simulink model "inverter_s2_kal"  (R2023b)
settings: Solver=ode15s  StartTime=0.0  StopTime=0.1  MaxStep=sim_max_step  RelTol=sim_rel_tol  AbsTol=sim_abs_tol  EnableMultiTasking=on
PreLoadFcn:
  | d08_pre_dir = fileparts(which('inverter_s2_kal')); if isempty(d08_pre_dir), d08_pre_dir = pwd; end; run(fullfile(d08_pre_dir, 'inverter_common_parameters.m')); clear d08_pre_dir
InitFcn:
  | run(fullfile(fileparts(get_param(bdroot,'FileName')),'inverter_common_parameters.m'));
  | kal_dosya = fullfile(fileparts(get_param(bdroot,'FileName')), [bdroot '_kalibrasyon.m']); if isfile(kal_dosya), run(kal_dosya); end; clear kal_dosya
values from neighbouring files (symbols this model uses):
  EMC_k = EMC_M/EMC_Lw    (= 0.995)    [inverter_common_parameters.m]
  EMC_Rcore = 1e5    (= 100000)    [inverter_common_parameters.m]
  EMC_Rw = 5e-3    (= 0.005)    [inverter_common_parameters.m]
  f_grid = 50    [inverter_common_parameters.m]
  K11 = 0.7865    [inverter_common_parameters.m]    (also in inverter_s1_kal_kalibrasyon.m = 0.7865023595)
  K12 = 0.79400    (= 0.794)    [inverter_common_parameters.m]    (also in inverter_s2_kal_kalibrasyon.m = 0.7679568)
  L1_core_Rp = 600    [inverter_common_parameters.m]
  measurement_gain = 20    [inverter_common_parameters.m]
  phase_deg1 = -0.44    [inverter_common_parameters.m]    (also in inverter_s1_kal_kalibrasyon.m = -0.36607)
  phase_deg2 = 0    [inverter_common_parameters.m]    (also in inverter_s2_kal_kalibrasyon.m = 0.1121)
  pwm_ref_amp = 1    [inverter_common_parameters.m]
  pwm_ref_Ts = 1e-6    (= 1e-06)    [inverter_common_parameters.m]
  R_bleed_1 = 220e3    (= 220000)    [inverter_common_parameters.m]
  R_bleed_2 = 220e3    (= 220000)    [inverter_common_parameters.m]
  Rdc = 1e-3    (= 0.001)    [inverter_common_parameters.m]
libraries: ee_lib x64, fl_lib x54, nesl_utility x30, spsOnDelayLib x12, spsMeanLib x10, spsPWMGeneratorDCDCLib x6, spsTHDLib x4, eePowerMeasurement x2, spsPowerLib x2, spsRMSLib x2, spspowerguiLib x1
(part 3 of 3)

== system inverter_s2_kal/AC Current Sensor1 ==
  Current Sensor : fl_lib/Electrical/Electrical Sensors/Current Sensor
  PS-Simulink Converter : nesl_utility/PS-Simulink Converter  PhysicalDomain=network_engine_domain  SubClassName=ps_output  LeftPortType=input  RightPortType=output  PseudoPeriodic=off  Frequencies=[]  VectorFormat=1-D array  Unit=1  AffineConversion=off
  + : PMIOPort  Side=Right
  - : PMIOPort  Port=2  Side=Right
  tag scope: i_ac1=global
  wires:
  PS-Simulink Converter/1 -> [i_ac1]
  connections:
  Current Sensor/RConn1 -- PS-Simulink Converter/LConn1
  +/RConn1 -- Current Sensor/LConn1
  Current Sensor/RConn2 -- -/RConn1

== system inverter_s2_kal/AC Current Sensor2 ==
  Current Sensor : fl_lib/Electrical/Electrical Sensors/Current Sensor
  PS-Simulink Converter : nesl_utility/PS-Simulink Converter  PhysicalDomain=network_engine_domain  SubClassName=ps_output  LeftPortType=input  RightPortType=output  PseudoPeriodic=off  Frequencies=[]  VectorFormat=1-D array  Unit=1  AffineConversion=off
  + : PMIOPort  Side=Right
  - : PMIOPort  Port=2  Side=Right
  tag scope: i_ac2=global
  wires:
  PS-Simulink Converter/1 -> [i_ac2]
  connections:
  Current Sensor/RConn1 -- PS-Simulink Converter/LConn1
  +/RConn1 -- Current Sensor/LConn1
  Current Sensor/RConn2 -- -/RConn1

== system inverter_s2_kal/AC Voltage Sensor1 ==
  PS-Simulink Converter : nesl_utility/PS-Simulink Converter  PhysicalDomain=network_engine_domain  SubClassName=ps_output  LeftPortType=input  RightPortType=output  PseudoPeriodic=off  Frequencies=[]  VectorFormat=1-D array  Unit=1  AffineConversion=off
  Voltage Sensor : fl_lib/Electrical/Electrical Sensors/Voltage Sensor
  - : PMIOPort  Side=Left
  + : PMIOPort  Port=2  Side=Right
  tag scope: v_ac1=global
  wires:
  PS-Simulink Converter/1 -> [v_ac1]
  connections:
  Voltage Sensor/RConn2 -- -/RConn1
  Voltage Sensor/RConn1 -- PS-Simulink Converter/LConn1
  Voltage Sensor/LConn1 -- +/RConn1

== system inverter_s2_kal/AC Voltage Sensor2 ==
  PS-Simulink Converter : nesl_utility/PS-Simulink Converter  PhysicalDomain=network_engine_domain  SubClassName=ps_output  LeftPortType=input  RightPortType=output  PseudoPeriodic=off  Frequencies=[]  VectorFormat=1-D array  Unit=1  AffineConversion=off
  Voltage Sensor : fl_lib/Electrical/Electrical Sensors/Voltage Sensor
  - : PMIOPort  Side=Left
  + : PMIOPort  Port=2  Side=Right
  tag scope: v_inv1=global
  wires:
  PS-Simulink Converter/1 -> [v_inv1]
  connections:
  Voltage Sensor/LConn1 -- +/RConn1
  Voltage Sensor/RConn1 -- PS-Simulink Converter/LConn1
  Voltage Sensor/RConn2 -- -/RConn1

== system inverter_s2_kal/AC Voltage Sensor3 ==
  PS-Simulink Converter : nesl_utility/PS-Simulink Converter  PhysicalDomain=network_engine_domain  SubClassName=ps_output  LeftPortType=input  RightPortType=output  PseudoPeriodic=off  Frequencies=[]  VectorFormat=1-D array  Unit=1  AffineConversion=off
  Voltage Sensor : fl_lib/Electrical/Electrical Sensors/Voltage Sensor
  - : PMIOPort  Side=Left
  + : PMIOPort  Port=2  Side=Right
  tag scope: v_ac2=global
  wires:
  PS-Simulink Converter/1 -> [v_ac2]
  connections:
  Voltage Sensor/RConn2 -- -/RConn1
  Voltage Sensor/RConn1 -- PS-Simulink Converter/LConn1
  Voltage Sensor/LConn1 -- +/RConn1

== system inverter_s2_kal/AC Voltage Sensor4 ==
  PS-Simulink Converter : nesl_utility/PS-Simulink Converter  PhysicalDomain=network_engine_domain  SubClassName=ps_output  LeftPortType=input  RightPortType=output  PseudoPeriodic=off  Frequencies=[]  VectorFormat=1-D array  Unit=1  AffineConversion=off
  Voltage Sensor : fl_lib/Electrical/Electrical Sensors/Voltage Sensor
  - : PMIOPort  Side=Left
  + : PMIOPort  Port=2  Side=Right
  tag scope: v_inv2=global
  wires:
  PS-Simulink Converter/1 -> [v_inv2]
  connections:
  Voltage Sensor/LConn1 -- +/RConn1
  Voltage Sensor/RConn1 -- PS-Simulink Converter/LConn1
  Voltage Sensor/RConn2 -- -/RConn1

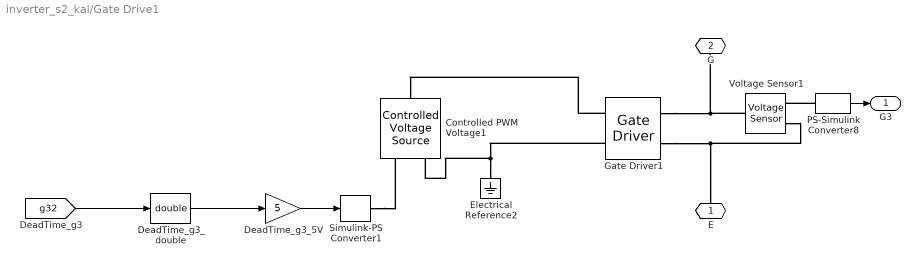
== system inverter_s2_kal/Gate Drive1 ==
  Controlled PWM Voltage1 : fl_lib/Electrical/Electrical Sources/Controlled Voltage Source
  DeadTime_g3_5V : Gain  Gain=5  OutDataTypeStr=double
  DeadTime_g3_double : DataTypeConversion  OutDataTypeStr=double  SaturateOnIntegerOverflow=off  RndMeth=Floor
  Electrical Reference2 : fl_lib/Electrical/Electrical Elements/Electrical Reference
  Gate Driver1 : ee_lib/Semiconductors & Converters/Gate Driver  port_option=ee.enum.controlport.elec  uHigh=4 V  uLow=3 V  uHighValue=gate_logic_high  uLowValue=gate_logic_low  vHigh=Vgate_on V  vLow=Vgate_off V  tHigh=gate_driver_ton s  tLow=gate_driver_toff s  parameterization=1  rHigh=RG_total Ohm  rLow=RG_total Ohm  tRise=gate_driver_rise s  tFall=gate_driver_fall s  cLoad=gate_driver_cload F  enable_faults=0  t_fault=1 s  fault_type=1  ZonTime_specify=off  ZonTime_priority=None  ZonTime=0 s  ZoffTime_specify=off  ZoffTime_priority=None  ZoffTime=0 s
  PS-Simulink Converter8 : nesl_utility/PS-Simulink Converter  PhysicalDomain=network_engine_domain  SubClassName=ps_output  LeftPortType=input  RightPortType=output  PseudoPeriodic=off  Frequencies=[]  VectorFormat=1-D array  Unit=1  AffineConversion=off
  Simulink-PS Converter1 : nesl_utility/Simulink-PS Converter  PhysicalDomain=network_engine_domain  SubClassName=ps_input  LeftPortType=input  RightPortType=output  PseudoPeriodic=off  Frequencies=[]  NoiseDistribution=none  NoiseParameters=[]  Unit=V  AffineConversion=off  FilteringAndDerivatives=filter  SimscapeFilterOrder=1  InputFilterTimeConstant=1e-7  UdotUserProvided=1
  Voltage Sensor1 : fl_lib/Electrical/Electrical Sensors/Voltage Sensor
  E : PMIOPort  Side=Right
  G : PMIOPort  Port=2  Side=Right
  G3 : Outport  VectorParamsAs1DForOutWhenUnconnected=off
  wires:
  PS-Simulink Converter8/1 -> G3/1
  [g32] -> DeadTime_g3_double/1
  DeadTime_g3_double/1 -> DeadTime_g3_5V/1
  DeadTime_g3_5V/1 -> Simulink-PS Converter1/1
  connections:
  Gate Driver1/RConn2 -- Voltage Sensor1/RConn2 -- E/RConn1
  Gate Driver1/RConn1 -- Voltage Sensor1/LConn1 -- G/RConn1
  PS-Simulink Converter8/LConn1 -- Voltage Sensor1/RConn1
  Gate Driver1/LConn2 -- Electrical Reference2/LConn1 -- Controlled PWM Voltage1/RConn2
  Simulink-PS Converter1/RConn1 -- Controlled PWM Voltage1/RConn1
  Gate Driver1/LConn1 -- Controlled PWM Voltage1/LConn1

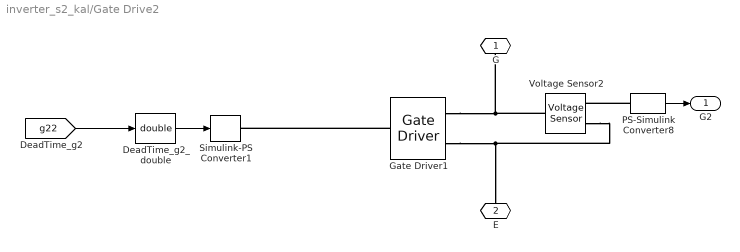
== system inverter_s2_kal/Gate Drive2 ==
  DeadTime_g2_double : DataTypeConversion  OutDataTypeStr=double  SaturateOnIntegerOverflow=off  RndMeth=Floor
  Gate Driver1 : ee_lib/Semiconductors & Converters/Gate Driver  port_option=ee.enum.controlport.ps  uHigh=4 V  uLow=3 V  uHighValue=gate_logic_high  uLowValue=gate_logic_low  vHigh=Vgate_on V  vLow=Vgate_off V  tHigh=gate_driver_ton s  tLow=gate_driver_toff s  parameterization=1  rHigh=RG_total Ohm  rLow=RG_total Ohm  tRise=gate_driver_rise s  tFall=gate_driver_fall s  cLoad=gate_driver_cload F  enable_faults=0  t_fault=1 s  fault_type=1  ZonTime_specify=off  ZonTime_priority=None  ZonTime=0 s  ZoffTime_specify=off  ZoffTime_priority=None  ZoffTime=0 s
      settings: InternalSimscapePortConfiguration="{\"Bottom\":[],\"Left\":[{\"id\":\"u\",\"label\":\"u\",\"type\":\"input\"}],\"Right\":[{\"id\":\"G\",\"label\":\"G\",\"type\":\"foundation.electrical.electrical\"},{\"id\":\"S\",\"label\":\"S\",\"type\":\"foundation.electrical.electrical\"}],\"Top\":[]}"
  PS-Simulink Converter8 : nesl_utility/PS-Simulink Converter  PhysicalDomain=network_engine_domain  SubClassName=ps_output  LeftPortType=input  RightPortType=output  PseudoPeriodic=off  Frequencies=[]  VectorFormat=1-D array  Unit=1  AffineConversion=off
  Simulink-PS Converter1 : nesl_utility/Simulink-PS Converter  PhysicalDomain=network_engine_domain  SubClassName=ps_input  LeftPortType=input  RightPortType=output  PseudoPeriodic=off  Frequencies=[]  NoiseDistribution=none  NoiseParameters=[]  Unit=1  AffineConversion=off  FilteringAndDerivatives=filter  SimscapeFilterOrder=1  InputFilterTimeConstant=1e-7  UdotUserProvided=1
  Voltage Sensor2 : fl_lib/Electrical/Electrical Sensors/Voltage Sensor
  G : PMIOPort  Side=Right
  E : PMIOPort  Port=2  Side=Right
  G2 : Outport  VectorParamsAs1DForOutWhenUnconnected=off
  wires:
  PS-Simulink Converter8/1 -> G2/1
  [g22] -> DeadTime_g2_double/1
  DeadTime_g2_double/1 -> Simulink-PS Converter1/1
  connections:
  Gate Driver1/RConn2 -- Voltage Sensor2/RConn2 -- E/RConn1
  Gate Driver1/RConn1 -- Voltage Sensor2/LConn1 -- G/RConn1
  PS-Simulink Converter8/LConn1 -- Voltage Sensor2/RConn1
  Gate Driver1/LConn1 -- Simulink-PS Converter1/RConn1

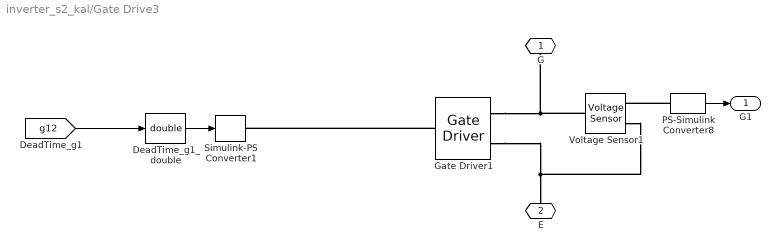
== system inverter_s2_kal/Gate Drive3 ==
  DeadTime_g1_double : DataTypeConversion  OutDataTypeStr=double  SaturateOnIntegerOverflow=off  RndMeth=Floor
  Gate Driver1 : ee_lib/Semiconductors & Converters/Gate Driver  port_option=ee.enum.controlport.ps  uHigh=4 V  uLow=3 V  uHighValue=gate_logic_high  uLowValue=gate_logic_low  vHigh=Vgate_on V  vLow=Vgate_off V  tHigh=gate_driver_ton s  tLow=gate_driver_toff s  parameterization=1  rHigh=RG_total Ohm  rLow=RG_total Ohm  tRise=gate_driver_rise s  tFall=gate_driver_fall s  cLoad=gate_driver_cload F  enable_faults=0  t_fault=1 s  fault_type=1  ZonTime_specify=off  ZonTime_priority=None  ZonTime=0 s  ZoffTime_specify=off  ZoffTime_priority=None  ZoffTime=0 s
      settings: InternalSimscapePortConfiguration="{\"Bottom\":[],\"Left\":[{\"id\":\"u\",\"label\":\"u\",\"type\":\"input\"}],\"Right\":[{\"id\":\"G\",\"label\":\"G\",\"type\":\"foundation.electrical.electrical\"},{\"id\":\"S\",\"label\":\"S\",\"type\":\"foundation.electrical.electrical\"}],\"Top\":[]}"
  PS-Simulink Converter8 : nesl_utility/PS-Simulink Converter  PhysicalDomain=network_engine_domain  SubClassName=ps_output  LeftPortType=input  RightPortType=output  PseudoPeriodic=off  Frequencies=[]  VectorFormat=1-D array  Unit=1  AffineConversion=off
  Simulink-PS Converter1 : nesl_utility/Simulink-PS Converter  PhysicalDomain=network_engine_domain  SubClassName=ps_input  LeftPortType=input  RightPortType=output  PseudoPeriodic=off  Frequencies=[]  NoiseDistribution=none  NoiseParameters=[]  Unit=1  AffineConversion=off  FilteringAndDerivatives=filter  SimscapeFilterOrder=1  InputFilterTimeConstant=1e-7  UdotUserProvided=1
  Voltage Sensor1 : fl_lib/Electrical/Electrical Sensors/Voltage Sensor
  G : PMIOPort  Side=Right
  E : PMIOPort  Port=2  Side=Right
  G1 : Outport  VectorParamsAs1DForOutWhenUnconnected=off
  wires:
  PS-Simulink Converter8/1 -> G1/1
  [g12] -> DeadTime_g1_double/1
  DeadTime_g1_double/1 -> Simulink-PS Converter1/1
  connections:
  Gate Driver1/RConn1 -- G/RConn1 -- Voltage Sensor1/LConn1
  Gate Driver1/RConn2 -- Voltage Sensor1/RConn2 -- E/RConn1
  PS-Simulink Converter8/LConn1 -- Voltage Sensor1/RConn1
  Gate Driver1/LConn1 -- Simulink-PS Converter1/RConn1

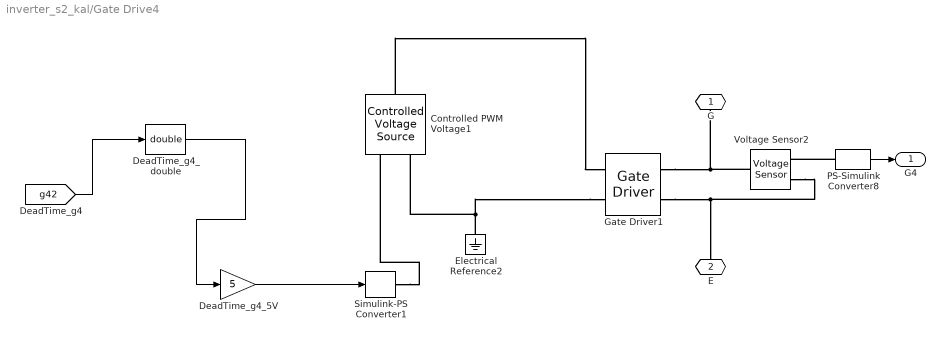
== system inverter_s2_kal/Gate Drive4 ==
  Controlled PWM Voltage1 : fl_lib/Electrical/Electrical Sources/Controlled Voltage Source
  DeadTime_g4_5V : Gain  Gain=5  OutDataTypeStr=double
  DeadTime_g4_double : DataTypeConversion  OutDataTypeStr=double  SaturateOnIntegerOverflow=off  RndMeth=Floor
  Electrical Reference2 : fl_lib/Electrical/Electrical Elements/Electrical Reference
  Gate Driver1 : ee_lib/Semiconductors & Converters/Gate Driver  port_option=ee.enum.controlport.elec  uHigh=4 V  uLow=3 V  uHighValue=gate_logic_high  uLowValue=gate_logic_low  vHigh=Vgate_on V  vLow=Vgate_off V  tHigh=gate_driver_ton s  tLow=gate_driver_toff s  parameterization=1  rHigh=RG_total Ohm  rLow=RG_total Ohm  tRise=gate_driver_rise s  tFall=gate_driver_fall s  cLoad=gate_driver_cload F  enable_faults=0  t_fault=1 s  fault_type=1  ZonTime_specify=off  ZonTime_priority=None  ZonTime=0 s  ZoffTime_specify=off  ZoffTime_priority=None  ZoffTime=0 s
  PS-Simulink Converter8 : nesl_utility/PS-Simulink Converter  PhysicalDomain=network_engine_domain  SubClassName=ps_output  LeftPortType=input  RightPortType=output  PseudoPeriodic=off  Frequencies=[]  VectorFormat=1-D array  Unit=1  AffineConversion=off
  Simulink-PS Converter1 : nesl_utility/Simulink-PS Converter  PhysicalDomain=network_engine_domain  SubClassName=ps_input  LeftPortType=input  RightPortType=output  PseudoPeriodic=off  Frequencies=[]  NoiseDistribution=none  NoiseParameters=[]  Unit=V  AffineConversion=off  FilteringAndDerivatives=filter  SimscapeFilterOrder=1  InputFilterTimeConstant=1e-7  UdotUserProvided=1
  Voltage Sensor2 : fl_lib/Electrical/Electrical Sensors/Voltage Sensor
  G : PMIOPort  Side=Right
  E : PMIOPort  Port=2  Side=Right
  G4 : Outport  VectorParamsAs1DForOutWhenUnconnected=off
  wires:
  PS-Simulink Converter8/1 -> G4/1
  [g42] -> DeadTime_g4_double/1
  DeadTime_g4_double/1 -> DeadTime_g4_5V/1
  DeadTime_g4_5V/1 -> Simulink-PS Converter1/1
  connections:
  Gate Driver1/LConn2 -- Electrical Reference2/LConn1 -- Controlled PWM Voltage1/RConn2
  Gate Driver1/RConn1 -- Voltage Sensor2/LConn1 -- G/RConn1
  Gate Driver1/RConn2 -- E/RConn1 -- Voltage Sensor2/RConn2
  PS-Simulink Converter8/LConn1 -- Voltage Sensor2/RConn1
  Simulink-PS Converter1/RConn1 -- Controlled PWM Voltage1/RConn1
  Controlled PWM Voltage1/LConn1 -- Gate Driver1/LConn1

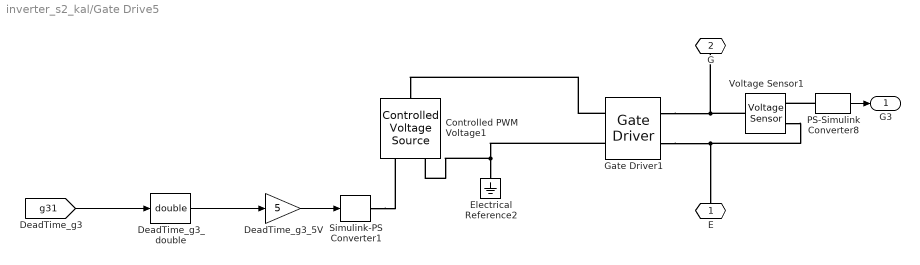
== system inverter_s2_kal/Gate Drive5 ==
  Controlled PWM Voltage1 : fl_lib/Electrical/Electrical Sources/Controlled Voltage Source
  DeadTime_g3_5V : Gain  Gain=5  OutDataTypeStr=double
  DeadTime_g3_double : DataTypeConversion  OutDataTypeStr=double  SaturateOnIntegerOverflow=off  RndMeth=Floor
  Electrical Reference2 : fl_lib/Electrical/Electrical Elements/Electrical Reference
  Gate Driver1 : ee_lib/Semiconductors & Converters/Gate Driver  port_option=ee.enum.controlport.elec  uHigh=4 V  uLow=3 V  uHighValue=gate_logic_high  uLowValue=gate_logic_low  vHigh=Vgate_on V  vLow=Vgate_off V  tHigh=gate_driver_ton s  tLow=gate_driver_toff s  parameterization=1  rHigh=RG_total Ohm  rLow=RG_total Ohm  tRise=gate_driver_rise s  tFall=gate_driver_fall s  cLoad=gate_driver_cload F  enable_faults=0  t_fault=1 s  fault_type=1  ZonTime_specify=off  ZonTime_priority=None  ZonTime=0 s  ZoffTime_specify=off  ZoffTime_priority=None  ZoffTime=0 s
  PS-Simulink Converter8 : nesl_utility/PS-Simulink Converter  PhysicalDomain=network_engine_domain  SubClassName=ps_output  LeftPortType=input  RightPortType=output  PseudoPeriodic=off  Frequencies=[]  VectorFormat=1-D array  Unit=1  AffineConversion=off
  Simulink-PS Converter1 : nesl_utility/Simulink-PS Converter  PhysicalDomain=network_engine_domain  SubClassName=ps_input  LeftPortType=input  RightPortType=output  PseudoPeriodic=off  Frequencies=[]  NoiseDistribution=none  NoiseParameters=[]  Unit=V  AffineConversion=off  FilteringAndDerivatives=filter  SimscapeFilterOrder=1  InputFilterTimeConstant=1e-7  UdotUserProvided=1
  Voltage Sensor1 : fl_lib/Electrical/Electrical Sensors/Voltage Sensor
  E : PMIOPort  Side=Right
  G : PMIOPort  Port=2  Side=Right
  G3 : Outport  VectorParamsAs1DForOutWhenUnconnected=off
  wires:
  PS-Simulink Converter8/1 -> G3/1
  [g31] -> DeadTime_g3_double/1
  DeadTime_g3_double/1 -> DeadTime_g3_5V/1
  DeadTime_g3_5V/1 -> Simulink-PS Converter1/1
  connections:
  Gate Driver1/RConn2 -- Voltage Sensor1/RConn2 -- E/RConn1
  Gate Driver1/RConn1 -- Voltage Sensor1/LConn1 -- G/RConn1
  PS-Simulink Converter8/LConn1 -- Voltage Sensor1/RConn1
  Gate Driver1/LConn2 -- Electrical Reference2/LConn1 -- Controlled PWM Voltage1/RConn2
  Simulink-PS Converter1/RConn1 -- Controlled PWM Voltage1/RConn1
  Gate Driver1/LConn1 -- Controlled PWM Voltage1/LConn1

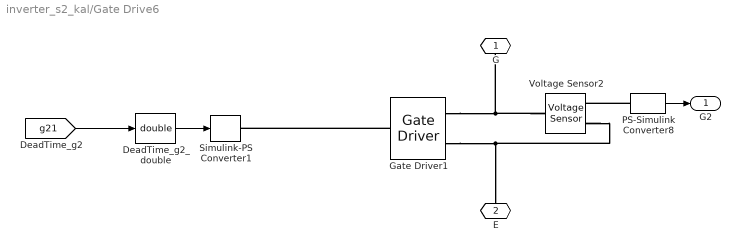
== system inverter_s2_kal/Gate Drive6 ==
  DeadTime_g2_double : DataTypeConversion  OutDataTypeStr=double  SaturateOnIntegerOverflow=off  RndMeth=Floor
  Gate Driver1 : ee_lib/Semiconductors & Converters/Gate Driver  port_option=ee.enum.controlport.ps  uHigh=4 V  uLow=3 V  uHighValue=gate_logic_high  uLowValue=gate_logic_low  vHigh=Vgate_on V  vLow=Vgate_off V  tHigh=gate_driver_ton s  tLow=gate_driver_toff s  parameterization=1  rHigh=RG_total Ohm  rLow=RG_total Ohm  tRise=gate_driver_rise s  tFall=gate_driver_fall s  cLoad=gate_driver_cload F  enable_faults=0  t_fault=1 s  fault_type=1  ZonTime_specify=off  ZonTime_priority=None  ZonTime=0 s  ZoffTime_specify=off  ZoffTime_priority=None  ZoffTime=0 s
      settings: InternalSimscapePortConfiguration="{\"Bottom\":[],\"Left\":[{\"id\":\"u\",\"label\":\"u\",\"type\":\"input\"}],\"Right\":[{\"id\":\"G\",\"label\":\"G\",\"type\":\"foundation.electrical.electrical\"},{\"id\":\"S\",\"label\":\"S\",\"type\":\"foundation.electrical.electrical\"}],\"Top\":[]}"
  PS-Simulink Converter8 : nesl_utility/PS-Simulink Converter  PhysicalDomain=network_engine_domain  SubClassName=ps_output  LeftPortType=input  RightPortType=output  PseudoPeriodic=off  Frequencies=[]  VectorFormat=1-D array  Unit=1  AffineConversion=off
  Simulink-PS Converter1 : nesl_utility/Simulink-PS Converter  PhysicalDomain=network_engine_domain  SubClassName=ps_input  LeftPortType=input  RightPortType=output  PseudoPeriodic=off  Frequencies=[]  NoiseDistribution=none  NoiseParameters=[]  Unit=1  AffineConversion=off  FilteringAndDerivatives=filter  SimscapeFilterOrder=1  InputFilterTimeConstant=1e-7  UdotUserProvided=1
  Voltage Sensor2 : fl_lib/Electrical/Electrical Sensors/Voltage Sensor
  G : PMIOPort  Side=Right
  E : PMIOPort  Port=2  Side=Right
  G2 : Outport  VectorParamsAs1DForOutWhenUnconnected=off
  wires:
  PS-Simulink Converter8/1 -> G2/1
  [g21] -> DeadTime_g2_double/1
  DeadTime_g2_double/1 -> Simulink-PS Converter1/1
  connections:
  Gate Driver1/RConn2 -- Voltage Sensor2/RConn2 -- E/RConn1
  Gate Driver1/RConn1 -- Voltage Sensor2/LConn1 -- G/RConn1
  PS-Simulink Converter8/LConn1 -- Voltage Sensor2/RConn1
  Gate Driver1/LConn1 -- Simulink-PS Converter1/RConn1

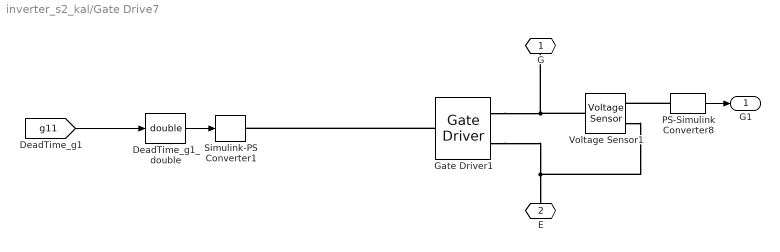
== system inverter_s2_kal/Gate Drive7 ==
  DeadTime_g1_double : DataTypeConversion  OutDataTypeStr=double  SaturateOnIntegerOverflow=off  RndMeth=Floor
  Gate Driver1 : ee_lib/Semiconductors & Converters/Gate Driver  port_option=ee.enum.controlport.ps  uHigh=4 V  uLow=3 V  uHighValue=gate_logic_high  uLowValue=gate_logic_low  vHigh=Vgate_on V  vLow=Vgate_off V  tHigh=gate_driver_ton s  tLow=gate_driver_toff s  parameterization=1  rHigh=RG_total Ohm  rLow=RG_total Ohm  tRise=gate_driver_rise s  tFall=gate_driver_fall s  cLoad=gate_driver_cload F  enable_faults=0  t_fault=1 s  fault_type=1  ZonTime_specify=off  ZonTime_priority=None  ZonTime=0 s  ZoffTime_specify=off  ZoffTime_priority=None  ZoffTime=0 s
      settings: InternalSimscapePortConfiguration="{\"Bottom\":[],\"Left\":[{\"id\":\"u\",\"label\":\"u\",\"type\":\"input\"}],\"Right\":[{\"id\":\"G\",\"label\":\"G\",\"type\":\"foundation.electrical.electrical\"},{\"id\":\"S\",\"label\":\"S\",\"type\":\"foundation.electrical.electrical\"}],\"Top\":[]}"
  PS-Simulink Converter8 : nesl_utility/PS-Simulink Converter  PhysicalDomain=network_engine_domain  SubClassName=ps_output  LeftPortType=input  RightPortType=output  PseudoPeriodic=off  Frequencies=[]  VectorFormat=1-D array  Unit=1  AffineConversion=off
  Simulink-PS Converter1 : nesl_utility/Simulink-PS Converter  PhysicalDomain=network_engine_domain  SubClassName=ps_input  LeftPortType=input  RightPortType=output  PseudoPeriodic=off  Frequencies=[]  NoiseDistribution=none  NoiseParameters=[]  Unit=1  AffineConversion=off  FilteringAndDerivatives=filter  SimscapeFilterOrder=1  InputFilterTimeConstant=1e-7  UdotUserProvided=1
  Voltage Sensor1 : fl_lib/Electrical/Electrical Sensors/Voltage Sensor
  G : PMIOPort  Side=Right
  E : PMIOPort  Port=2  Side=Right
  G1 : Outport  VectorParamsAs1DForOutWhenUnconnected=off
  wires:
  PS-Simulink Converter8/1 -> G1/1
  [g11] -> DeadTime_g1_double/1
  DeadTime_g1_double/1 -> Simulink-PS Converter1/1
  connections:
  Gate Driver1/RConn1 -- G/RConn1 -- Voltage Sensor1/LConn1
  Gate Driver1/RConn2 -- Voltage Sensor1/RConn2 -- E/RConn1
  PS-Simulink Converter8/LConn1 -- Voltage Sensor1/RConn1
  Gate Driver1/LConn1 -- Simulink-PS Converter1/RConn1

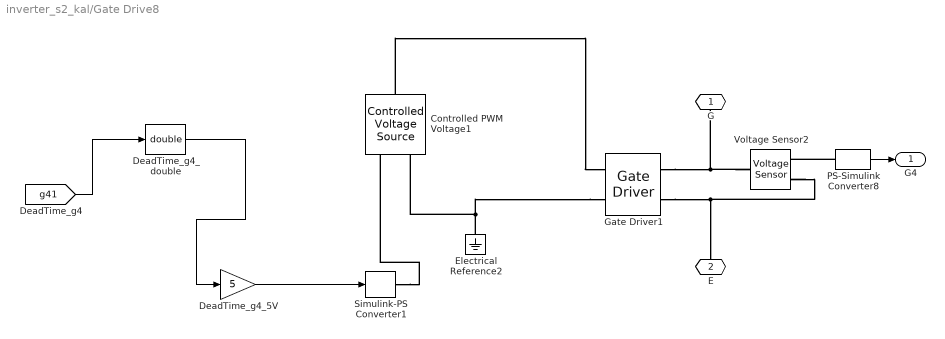
== system inverter_s2_kal/Gate Drive8 ==
  Controlled PWM Voltage1 : fl_lib/Electrical/Electrical Sources/Controlled Voltage Source
  DeadTime_g4_5V : Gain  Gain=5  OutDataTypeStr=double
  DeadTime_g4_double : DataTypeConversion  OutDataTypeStr=double  SaturateOnIntegerOverflow=off  RndMeth=Floor
  Electrical Reference2 : fl_lib/Electrical/Electrical Elements/Electrical Reference
  Gate Driver1 : ee_lib/Semiconductors & Converters/Gate Driver  port_option=ee.enum.controlport.elec  uHigh=4 V  uLow=3 V  uHighValue=gate_logic_high  uLowValue=gate_logic_low  vHigh=Vgate_on V  vLow=Vgate_off V  tHigh=gate_driver_ton s  tLow=gate_driver_toff s  parameterization=1  rHigh=RG_total Ohm  rLow=RG_total Ohm  tRise=gate_driver_rise s  tFall=gate_driver_fall s  cLoad=gate_driver_cload F  enable_faults=0  t_fault=1 s  fault_type=1  ZonTime_specify=off  ZonTime_priority=None  ZonTime=0 s  ZoffTime_specify=off  ZoffTime_priority=None  ZoffTime=0 s
  PS-Simulink Converter8 : nesl_utility/PS-Simulink Converter  PhysicalDomain=network_engine_domain  SubClassName=ps_output  LeftPortType=input  RightPortType=output  PseudoPeriodic=off  Frequencies=[]  VectorFormat=1-D array  Unit=1  AffineConversion=off
  Simulink-PS Converter1 : nesl_utility/Simulink-PS Converter  PhysicalDomain=network_engine_domain  SubClassName=ps_input  LeftPortType=input  RightPortType=output  PseudoPeriodic=off  Frequencies=[]  NoiseDistribution=none  NoiseParameters=[]  Unit=V  AffineConversion=off  FilteringAndDerivatives=filter  SimscapeFilterOrder=1  InputFilterTimeConstant=1e-7  UdotUserProvided=1
  Voltage Sensor2 : fl_lib/Electrical/Electrical Sensors/Voltage Sensor
  G : PMIOPort  Side=Right
  E : PMIOPort  Port=2  Side=Right
  G4 : Outport  VectorParamsAs1DForOutWhenUnconnected=off
  wires:
  PS-Simulink Converter8/1 -> G4/1
  [g41] -> DeadTime_g4_double/1
  DeadTime_g4_double/1 -> DeadTime_g4_5V/1
  DeadTime_g4_5V/1 -> Simulink-PS Converter1/1
  connections:
  Gate Driver1/LConn2 -- Electrical Reference2/LConn1 -- Controlled PWM Voltage1/RConn2
  Gate Driver1/RConn1 -- Voltage Sensor2/LConn1 -- G/RConn1
  Gate Driver1/RConn2 -- E/RConn1 -- Voltage Sensor2/RConn2
  PS-Simulink Converter8/LConn1 -- Voltage Sensor2/RConn1
  Simulink-PS Converter1/RConn1 -- Controlled PWM Voltage1/RConn1
  Controlled PWM Voltage1/LConn1 -- Gate Driver1/LConn1

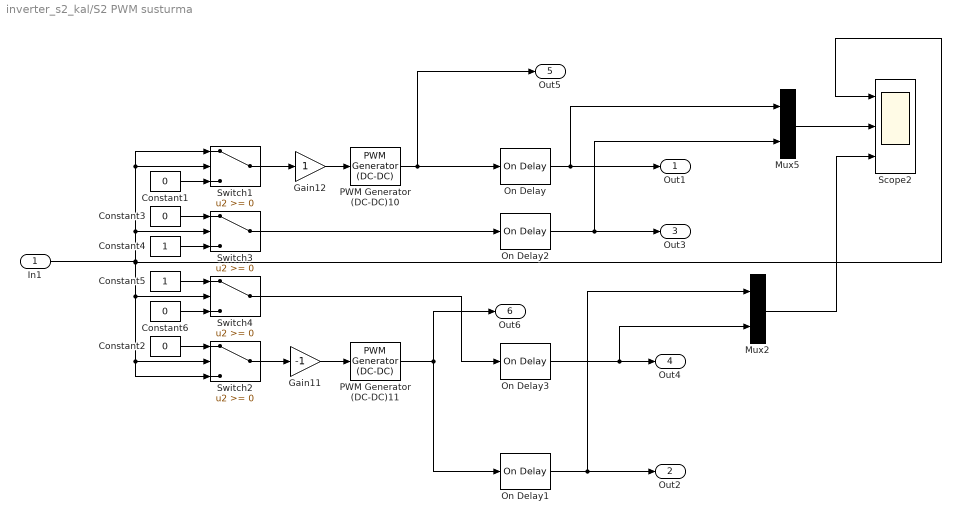
== system inverter_s2_kal/S2 PWM susturma ==
  In1 : Inport
  Constant{1..3,6} (4 alike) : Constant  Value=0
  Constant4 : Constant
  Constant5 : Constant
  Gain11 : Gain  Gain=-1
  Gain12 : Gain
  Mux2 : Mux  Inputs=2
  Mux5 : Mux  Inputs=2
  On Delay{,1..3} (4 alike) : spsOnDelayLib/On Delay  DelayType=On delay  delay=deadtime  ic=0  Ts=0
  PWM Generator (DC-DC)10 : spsPWMGeneratorDCDCLib/PWM Generator (DC-DC)  Fsw=fsw  Ts=1/fsw/100
  PWM Generator (DC-DC)11 : spsPWMGeneratorDCDCLib/PWM Generator (DC-DC)  Fsw=fsw  Ts=1/fsw/100
  Scope2 : Scope  NumInputPorts=3
  Switch{1..4} (4 alike) : Switch  SaturateOnIntegerOverflow=off  InputSameDT=off
  Out1 : Outport
  Out2 : Outport  Port=2
  Out3 : Outport  Port=3
  Out4 : Outport  Port=4
  Out5 : Outport  Port=5
  Out6 : Outport  Port=6
  wires:
  Mux2/1 -> Scope2/3
  Mux5/1 -> Scope2/2
  On Delay3/1 -> Out4/1, Mux2/2
  On Delay2/1 -> Out3/1, Mux5/2
  Switch3/1 -> On Delay2/1
  On Delay1/1 -> Out2/1, Mux2/1
  PWM Generator (DC-DC)11/1 -> On Delay1/1, Out6/1
  On Delay/1 -> Out1/1, Mux5/1
  PWM Generator (DC-DC)10/1 -> On Delay/1, Out5/1
  Gain12/1 -> PWM Generator (DC-DC)10/1
  Switch1/1 -> Gain12/1
  Constant2/1 -> Switch2/1
  Constant1/1 -> Switch1/3
  Switch2/1 -> Gain11/1
  Gain11/1 -> PWM Generator (DC-DC)11/1
  In1/1 -> Switch4/2, Switch2/2, Switch2/3, Scope2/1, Switch3/2, Switch1/2, Switch1/1
  Switch4/1 -> On Delay3/1
  Constant3/1 -> Switch3/1
  Constant4/1 -> Switch3/3
  Constant5/1 -> Switch4/1
  Constant6/1 -> Switch4/3

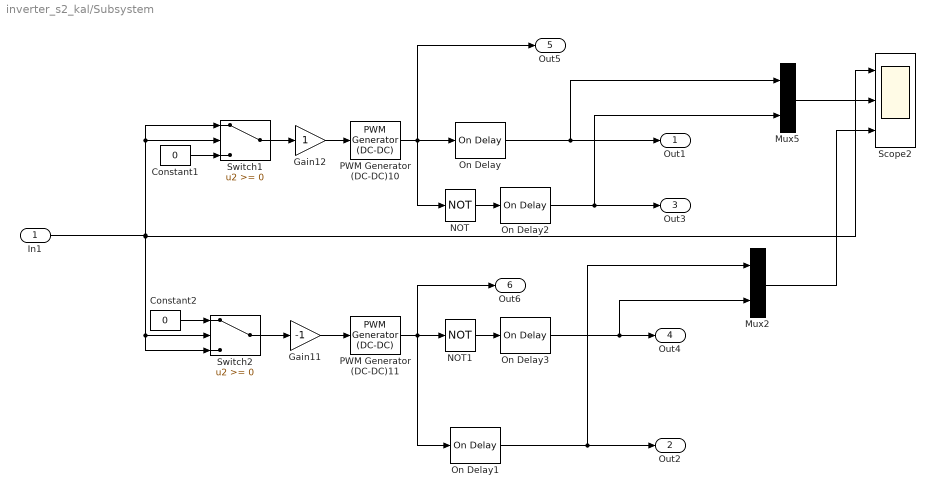
== system inverter_s2_kal/Subsystem ==
  In1 : Inport
  Constant1 : Constant  Value=0
  Constant2 : Constant  Value=0
  Gain11 : Gain  Gain=-1
  Gain12 : Gain
  Mux2 : Mux  Inputs=2
  Mux5 : Mux  Inputs=2
  NOT : Logic  Operator=NOT  IconShape=distinctive  AllPortsSameDT=off  OutDataTypeStr=boolean
  NOT1 : Logic  Operator=NOT  IconShape=distinctive  AllPortsSameDT=off  OutDataTypeStr=boolean
  On Delay{,1..3} (4 alike) : spsOnDelayLib/On Delay  DelayType=On delay  delay=deadtime  ic=0  Ts=0
  PWM Generator (DC-DC)10 : spsPWMGeneratorDCDCLib/PWM Generator (DC-DC)  Fsw=fsw  Ts=1/fsw/100
  PWM Generator (DC-DC)11 : spsPWMGeneratorDCDCLib/PWM Generator (DC-DC)  Fsw=fsw  Ts=1/fsw/100
  Scope2 : Scope  NumInputPorts=3
  Switch1 : Switch  SaturateOnIntegerOverflow=off  InputSameDT=off
  Switch2 : Switch  SaturateOnIntegerOverflow=off  InputSameDT=off
  Out1 : Outport
  Out2 : Outport  Port=2
  Out3 : Outport  Port=3
  Out4 : Outport  Port=4
  Out5 : Outport  Port=5
  Out6 : Outport  Port=6
  wires:
  Gain11/1 -> PWM Generator (DC-DC)11/1
  Switch2/1 -> Gain11/1
  Constant1/1 -> Switch1/3
  Constant2/1 -> Switch2/1
  Switch1/1 -> Gain12/1
  Gain12/1 -> PWM Generator (DC-DC)10/1
  PWM Generator (DC-DC)10/1 -> Out5/1, NOT/1, On Delay/1
  On Delay/1 -> Mux5/1, Out1/1
  PWM Generator (DC-DC)11/1 -> Out6/1, NOT1/1, On Delay1/1
  On Delay1/1 -> Mux2/1, Out2/1
  NOT/1 -> On Delay2/1
  On Delay2/1 -> Mux5/2, Out3/1
  NOT1/1 -> On Delay3/1
  On Delay3/1 -> Mux2/2, Out4/1
  In1/1 -> Switch1/1, Switch1/2, Scope2/1, Switch2/3, Switch2/2
  Mux5/1 -> Scope2/2
  Mux2/1 -> Scope2/3

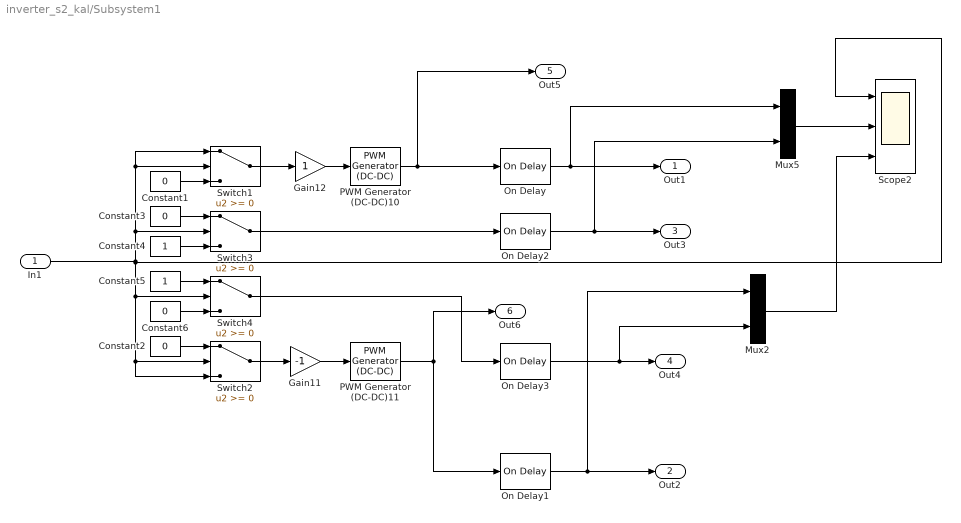
== system inverter_s2_kal/Subsystem1 ==
  In1 : Inport
  Constant{1..3,6} (4 alike) : Constant  Value=0
  Constant4 : Constant
  Constant5 : Constant
  Gain11 : Gain  Gain=-1
  Gain12 : Gain
  Mux2 : Mux  Inputs=2
  Mux5 : Mux  Inputs=2
  On Delay{,1..3} (4 alike) : spsOnDelayLib/On Delay  DelayType=On delay  delay=deadtime  ic=0  Ts=0
  PWM Generator (DC-DC)10 : spsPWMGeneratorDCDCLib/PWM Generator (DC-DC)  Fsw=fsw  Ts=1/fsw/100
  PWM Generator (DC-DC)11 : spsPWMGeneratorDCDCLib/PWM Generator (DC-DC)  Fsw=fsw  Ts=1/fsw/100
  Scope2 : Scope  NumInputPorts=3
  Switch{1..4} (4 alike) : Switch  SaturateOnIntegerOverflow=off  InputSameDT=off
  Out1 : Outport
  Out2 : Outport  Port=2
  Out3 : Outport  Port=3
  Out4 : Outport  Port=4
  Out5 : Outport  Port=5
  Out6 : Outport  Port=6
  wires:
  Mux2/1 -> Scope2/3
  Mux5/1 -> Scope2/2
  On Delay3/1 -> Out4/1, Mux2/2
  On Delay2/1 -> Out3/1, Mux5/2
  Switch3/1 -> On Delay2/1
  On Delay1/1 -> Out2/1, Mux2/1
  PWM Generator (DC-DC)11/1 -> On Delay1/1, Out6/1
  On Delay/1 -> Out1/1, Mux5/1
  PWM Generator (DC-DC)10/1 -> On Delay/1, Out5/1
  Gain12/1 -> PWM Generator (DC-DC)10/1
  Switch1/1 -> Gain12/1
  Constant2/1 -> Switch2/1
  Constant1/1 -> Switch1/3
  Switch2/1 -> Gain11/1
  Gain11/1 -> PWM Generator (DC-DC)11/1
  In1/1 -> Switch4/2, Switch2/2, Switch2/3, Scope2/1, Switch3/2, Switch1/2, Switch1/1
  Switch4/1 -> On Delay3/1
  Constant3/1 -> Switch3/1
  Constant4/1 -> Switch3/3
  Constant5/1 -> Switch4/1
  Constant6/1 -> Switch4/3
